simulink model "BESS_PV_WIND_STAGE2_R1_with_scopes_r2024b"  (R2024b)
settings: Solver=VariableStepAuto  StartTime=0.0  StopTime=10.0  RelTol=1e-3
InitFcn:
  | run(fullfile(fileparts(get_param(bdroot,'FileName')),'..','scripts','init_bess_pv_wind_stage2_r1.m'));
undefined symbols (not defined in the file): Control, G, S1, S2, S21, W1
libraries: ee_lib x27, nesl_utility x23, fl_lib x10, simulink x5
(part 1 of 2)
settings Model: Creator=fakebob2004  LastModifiedBy=fakebob2004
settings ModelReferenceCC: UpdateModelReferenceTargets=IfOutOfDate
settings ConfigComp: CovBoundaryAbsTol=1.0e-5
settings SimscapeCC: SimscapeNominalValues="[{\"value\":\"1\",\"unit\":\"A\"},{\"value\":\"1\",\"unit\":\"bar\"},{\"value\":\"1\",\"unit\":\"cm^2\"},{\"value\":\"1\",\"unit\":\"cm^3/s\"},{\"value\":\"1\",\"unit\":\"kJ/kg\"},{\"value\":\"1\",\"unit\":\"kW\"},{\"value\":\"1\",\"unit\":\"l\"},{\"value\":\"1\",\"unit\":\"N\"},{\"value\":\"1\",\"unit\":\"N*m\"},{\"value\":\"1\",\"unit\":\"V\"},{\"value\":\"0.001\",\"unit\":\"Wb\"}]"  SimscapeLogType=all  SimscapeLogDataHistory=10000

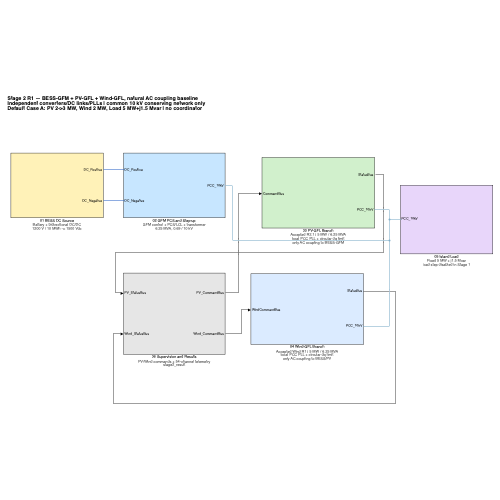
[thumbnail: Simulink's stored preview of the top-level diagram]
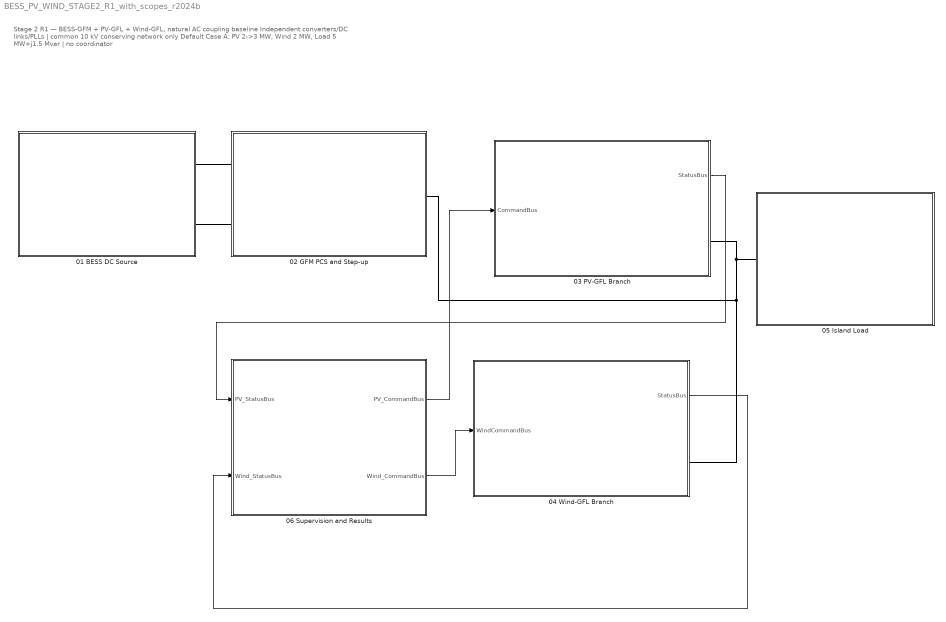
== system BESS_PV_WIND_STAGE2_R1_with_scopes_r2024b ==
  note: Stage 2 R1 — BESS-GFM + PV-GFL + Wind-GFL, natural AC coupling baseline
      | Independent converters/DC links/PLLs | common 10 kV conserving network only
      | Default Case A: PV 2->3 MW, Wind 2 MW, Load 5 MW+j1.5 Mvar | no coordinator
  01 BESS DC Source : Subsystem
      settings: AttributesFormatString=Battery + bidirectional DC/DC\n1200 V / 10 MWh -> 1500 Vdc
  02 GFM PCS and Step-up : Subsystem
      settings: AttributesFormatString=GFM control + PCS/LCL + transformer\n6.25 MVA, 0.69 / 10 kV
  03 PV-GFL Branch : Subsystem
      settings: AttributesFormatString=|
      | Accepted R2.1 | 5 MW / 6.25 MVA
      | local PCC PLL + circular dq limit
      | only AC coupling to BESS-GFM
  04 Wind-GFL Branch : Subsystem
      settings: AttributesFormatString=|
      | Accepted Wind R1 | 5 MW / 6.25 MVA
      | local PCC PLL + circular dq limit
      | only AC coupling to BESS/PV
  05 Island Load : Subsystem
      settings: AttributesFormatString=Fixed 5 MW + j1.5 Mvar\nload step disabled in Stage 1
  06 Supervision and Results : Subsystem
      settings: AttributesFormatString=PV/Wind commands + 54-channel telemetry\nstage2_result
  wires:
  06 Supervision and Results/1(PV_CommandBus) -> 03 PV-GFL Branch/1(CommandBus)
  03 PV-GFL Branch/1(StatusBus) -> 06 Supervision and Results/1(PV_StatusBus)
  06 Supervision and Results/2(Wind_CommandBus) -> 04 Wind-GFL Branch/1(WindCommandBus)
  04 Wind-GFL Branch/1(StatusBus) -> 06 Supervision and Results/2(Wind_StatusBus)
  connections:
  01 BESS DC Source/RConn1 -- 02 GFM PCS and Step-up/LConn1
  01 BESS DC Source/RConn2 -- 02 GFM PCS and Step-up/LConn2
  02 GFM PCS and Step-up/RConn1 -- 04 Wind-GFL Branch/RConn1 -- 05 Island Load/LConn1 -- 03 PV-GFL Branch/RConn1

== system BESS_PV_WIND_STAGE2_R1_with_scopes_r2024b/01 BESS DC Source ==
  01 Battery and DC Link : Subsystem
      settings: AttributesFormatString=1200 V / 10 MWh\n1500 V DC link
  02 Bidirectional DC-DC Control : Subsystem
      settings: AttributesFormatString=Vdc PI: 10 Hz\nIbat PI: 300 Hz
  DC_Positive : PMIOPort  Side=Right  ConnectionType=Connection: foundation.electrical.electrical
  DC_Negative : PMIOPort  Port=2  Side=Right  ConnectionType=Connection: foundation.electrical.electrical
  connections:
  01 Battery and DC Link/RConn1 -- DC_Negative/RConn1
  DC_Positive/RConn1 -- 01 Battery and DC Link/LConn1
  02 Bidirectional DC-DC Control/RConn1 -- 01 Battery and DC Link/LConn2

== system BESS_PV_WIND_STAGE2_R1_with_scopes_r2024b/02 GFM PCS and Step-up ==
  03 GFM Control and Limits : Subsystem
      settings: AttributesFormatString=P-f / Q-V / Virtual Z\nAC limit: 1.20 pu
  04 PCS Filter and Transformer : Subsystem
      settings: AttributesFormatString=6.25 MVA PCS + LCL\n0.69 / 10 kV transformer
  DC_Positive : PMIOPort  Side=Left  ConnectionType=Connection: foundation.electrical.electrical
  DC_Negative : PMIOPort  Port=2  Side=Left  ConnectionType=Connection: foundation.electrical.electrical
  PCC_10kV : PMIOPort  Port=3  Side=Right  ConnectionType=Connection: foundation.electrical.three_phase
  connections:
  04 PCS Filter and Transformer/RConn3 -- DC_Negative/RConn1
  04 PCS Filter and Transformer/RConn2 -- PCC_10kV/RConn1
  04 PCS Filter and Transformer/RConn1 -- DC_Positive/RConn1
  03 GFM Control and Limits/RConn1 -- 04 PCS Filter and Transformer/LConn1

== system BESS_PV_WIND_STAGE2_R1_with_scopes_r2024b/03 PV-GFL Branch ==
  CommandBus : Inport
  01 GFL PCS : Subsystem
  02 Step-up and PCC : Subsystem
  scope_R21_CurrentCommandBus : GotoTagVisibility  GotoTag=R21_CurrentCommandBus
  scope_R21_PCCMeasurementBus : GotoTagVisibility  GotoTag=R21_PCCMeasurementBus
  scope_R21_PrimaryMeasurementBus : GotoTagVisibility  GotoTag=R21_PrimaryMeasurementBus
  PCC_10kV : PMIOPort  Side=Right  ConnectionType=Connection: foundation.electrical.three_phase
  StatusBus : Outport
  wires:
  01 GFL PCS/1(StatusBus) -> StatusBus/1
  CommandBus/1 -> 01 GFL PCS/1(CommandBus)
  connections:
  01 GFL PCS/RConn1 -- 02 Step-up and PCC/LConn1
  02 Step-up and PCC/RConn1 -- PCC_10kV/RConn1

== system BESS_PV_WIND_STAGE2_R1_with_scopes_r2024b/04 Wind-GFL Branch ==
  WindCommandBus : Inport
  01 Aerodynamic and MPPT Available Power : Subsystem
  02 DC Energy Buffer and MSC Equivalent : Subsystem
  03 GFL PCS : Subsystem
  04 Step-up and PCC : Subsystem
  Wind StatusBus Elements : Mux  Inputs=2
  scope_WIND1_CurrentCommandBus : GotoTagVisibility  GotoTag=WIND1_CurrentCommandBus
  scope_WIND1_PCCMeasurementBus : GotoTagVisibility  GotoTag=WIND1_PCCMeasurementBus
  scope_WIND1_PrimaryMeasurementBus : GotoTagVisibility  GotoTag=WIND1_PrimaryMeasurementBus
  PCC_10kV : PMIOPort  Side=Right  ConnectionType=Connection: foundation.electrical.three_phase
  StatusBus : Outport
  wires:
  WindCommandBus/1 -> 01 Aerodynamic and MPPT Available Power/1(WindCommandBus)
  01 Aerodynamic and MPPT Available Power/1(WindSourceBus Out) -> 02 DC Energy Buffer and MSC Equivalent/1(WindSourceBus)
  Wind StatusBus Elements/1 -> StatusBus/1
  02 DC Energy Buffer and MSC Equivalent/1(PCS CommandBus Out) -> 03 GFL PCS/1(CommandBus)
  02 DC Energy Buffer and MSC Equivalent/2(Source StatusBus Out) -> Wind StatusBus Elements/2
  03 GFL PCS/1(StatusBus) -> Wind StatusBus Elements/1
  connections:
  04 Step-up and PCC/RConn1 -- PCC_10kV/RConn1
  03 GFL PCS/RConn1 -- 04 Step-up and PCC/LConn1

== system BESS_PV_WIND_STAGE2_R1_with_scopes_r2024b/05 Island Load ==
  Adjusted_Island_Load : ee_lib/Passive/Constant Power Load (Three-Phase)  port_option=ee.enum.threePhasePort.composite  FRated=G.f0_Hz Hz  active_power=S2.load.base_P_W W  reactive_power=S2.load.base_Q_var V*A  Vline_rms_min=0.70*G.ac.Vll_high_V V  tau=0.01 s  Vline_rms_ini=G.ac.Vll_high_V V  Vang_ini=0 deg  gmin=1e-6 S
  Load_Step_Command : Step  Time=G.load.step_time_s  Before=1  After=0  SampleTime=0
  Load_Step_to_PS : nesl_utility/Simulink-PS Converter  PhysicalDomain=network_engine_domain  SubClassName=ps_input  LeftPortType=input  RightPortType=output  PseudoPeriodic=off  Frequencies=[]  NoiseDistribution=none  NoiseParameters=[]  Unit=V  AffineConversion=off  FilteringAndDerivatives=zero  SimscapeFilterOrder=1  InputFilterTimeConstant=0.001  UdotUserProvided=0
  One_MW_Step_Load : ee_lib/Passive/Constant Power Load (Three-Phase)  port_option=ee.enum.threePhasePort.composite  FRated=G.f0_Hz Hz  active_power=0 W  reactive_power=0 V*A  Vline_rms_min=0.70*G.ac.Vll_high_V V  tau=0.01 s  Vline_rms_ini=G.ac.Vll_high_V V  Vang_ini=0 deg  gmin=1e-6 S
  Step_Load_Breaker : ee_lib/Switches & Breakers/Circuit Breaker (Three-Phase)  port_option=ee.enum.threePhasePort.composite  control_port_option=ee.enum.controlport.ps  R_closed=0.001 Ohm  G_open=1e-6 1/Ohm  threshold=0.5 V  breaker_behavior=ee.enum.switches.breakerBehavior.zeroCrossingEnable  i_th=1e-8 A
  PCC_10kV : PMIOPort  Side=Left  ConnectionType=Connection: foundation.electrical.three_phase
  tag scope: R8_05_Island_Load_Scenario_p1_signal=global
  wires:
  Load_Step_Command/1 -> Load_Step_to_PS/1, [R8_05_Island_Load_Scenario_p1_signal]  "step_breaker_cmd"
  connections:
  Step_Load_Breaker/RConn1 -- One_MW_Step_Load/LConn1
  PCC_10kV/RConn1 -- Adjusted_Island_Load/LConn1 -- Step_Load_Breaker/LConn2
  Load_Step_to_PS/RConn1 -- Step_Load_Breaker/LConn1

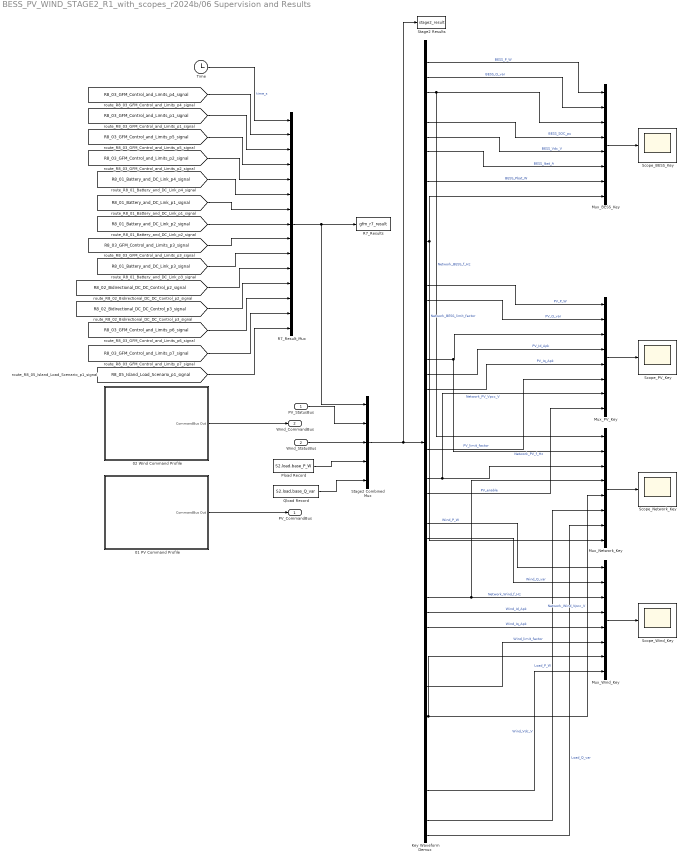
== system BESS_PV_WIND_STAGE2_R1_with_scopes_r2024b/06 Supervision and Results ==
  PV_StatusBus : Inport
  Wind_StatusBus : Inport  Port=2
  01 PV Command Profile : Subsystem
      settings: AttributesFormatString=|
      | CommandBus = [P*, Q*, enable]
      | commissioning scenario only
  02 Wind Command Profile : Subsystem
      settings: AttributesFormatString=|
      | WindCommandBus = [Pavailable, Pdispatch, Q, enable]
      | standalone commissioning scenario only
  Key Waveform Demux : Demux  Outputs=54
  Mux_BESS_Key : Mux  Inputs=8
  Mux_Network_Key : Mux  Inputs=8
  Mux_PV_Key : Mux  Inputs=8
  Mux_Wind_Key : Mux  Inputs=8
  Pload Record : Constant  Value=S2.load.base_P_W
  Qload Record : Constant  Value=S2.load.base_Q_var
  R7_Result_Mux : Mux  Inputs=15
  R7_Results : ToWorkspace  VariableName=gfm_r7_result  SampleTime=-1
  Scope_BESS_Key : Scope
  Scope_Network_Key : Scope
  Scope_PV_Key : Scope
  Scope_Wind_Key : Scope
  Stage2 Combined Mux : Mux  Inputs=5
  Stage2 Results : ToWorkspace  VariableName=stage2_result  SampleTime=-1
  Time : Clock
  PV_CommandBus : Outport
  Wind_CommandBus : Outport  Port=2
  wires:
  [R8_02_Bidirectional_DC_DC_Control_p3_signal] -> R7_Result_Mux/12
  [R8_03_GFM_Control_and_Limits_p4_signal] -> R7_Result_Mux/2
  [R8_01_Battery_and_DC_Link_p2_signal] -> R7_Result_Mux/8
  [R8_02_Bidirectional_DC_DC_Control_p2_signal] -> R7_Result_Mux/11
  [R8_03_GFM_Control_and_Limits_p3_signal] -> R7_Result_Mux/9
  [R8_01_Battery_and_DC_Link_p1_signal] -> R7_Result_Mux/7
  Time/1 -> R7_Result_Mux/1  "time_s"
  [R8_03_GFM_Control_and_Limits_p2_signal] -> R7_Result_Mux/5
  [R8_01_Battery_and_DC_Link_p4_signal] -> R7_Result_Mux/6
  [R8_01_Battery_and_DC_Link_p3_signal] -> R7_Result_Mux/10
  [R8_03_GFM_Control_and_Limits_p1_signal] -> R7_Result_Mux/3
  [R8_03_GFM_Control_and_Limits_p5_signal] -> R7_Result_Mux/4
  [R8_03_GFM_Control_and_Limits_p6_signal] -> R7_Result_Mux/13
  [R8_03_GFM_Control_and_Limits_p7_signal] -> R7_Result_Mux/14
  02 Wind Command Profile/1(CommandBus Out) -> Wind_CommandBus/1
  [R8_05_Island_Load_Scenario_p1_signal] -> R7_Result_Mux/15
  Key Waveform Demux/54 -> Mux_Network_Key/7  "Load_Q_var"
  Key Waveform Demux/46 -> Mux_Wind_Key/7, Mux_Network_Key/5  "Network_Wind_Vpcc_V"
  Key Waveform Demux/38 -> Mux_Wind_Key/3, Mux_Network_Key/4  "Network_Wind_f_Hz"
  01 PV Command Profile/1(CommandBus Out) -> PV_CommandBus/1
  Pload Record/1 -> Stage2 Combined Mux/4
  R7_Result_Mux/1 -> Stage2 Combined Mux/1, R7_Results/1
  Key Waveform Demux/39 -> Mux_Wind_Key/4  "Wind_Id_Apk"
  Key Waveform Demux/31 -> Mux_PV_Key/8  "PV_enable"
  PV_StatusBus/1 -> Stage2 Combined Mux/2
  Wind_StatusBus/1 -> Stage2 Combined Mux/3
  Qload Record/1 -> Stage2 Combined Mux/5
  Stage2 Combined Mux/1 -> Key Waveform Demux/1, Stage2 Results/1
  Key Waveform Demux/18 -> Mux_PV_Key/2  "PV_Q_var"
  Key Waveform Demux/10 -> Mux_BESS_Key/7  "BESS_Pbat_W"
  Key Waveform Demux/2 -> Mux_BESS_Key/1  "BESS_P_W"
  Key Waveform Demux/3 -> Mux_BESS_Key/2  "BESS_Q_var"
  Key Waveform Demux/28 -> Mux_PV_Key/6  "PV_limit_factor"
  Key Waveform Demux/4 -> Mux_BESS_Key/3, Mux_Network_Key/1  "Network_BESS_f_Hz"
  Key Waveform Demux/30 -> Mux_PV_Key/7, Mux_Network_Key/3  "Network_PV_Vpcc_V"
  Key Waveform Demux/22 -> Mux_PV_Key/3, Mux_Network_Key/2  "Network_PV_f_Hz"
  Key Waveform Demux/14 -> Mux_BESS_Key/8, Mux_Network_Key/8  "Network_BESS_limit_factor"
  Key Waveform Demux/6 -> Mux_BESS_Key/4  "BESS_SOC_pu"
  Key Waveform Demux/23 -> Mux_PV_Key/4  "PV_Id_Apk"
  Key Waveform Demux/7 -> Mux_BESS_Key/5  "BESS_Vdc_V"
  Key Waveform Demux/24 -> Mux_PV_Key/5  "PV_Iq_Apk"
  Key Waveform Demux/8 -> Mux_BESS_Key/6  "BESS_Ibat_A"
  Key Waveform Demux/17 -> Mux_PV_Key/1  "PV_P_W"
  Key Waveform Demux/33 -> Mux_Wind_Key/1  "Wind_P_W"
  Key Waveform Demux/34 -> Mux_Wind_Key/2  "Wind_Q_var"
  Key Waveform Demux/40 -> Mux_Wind_Key/5  "Wind_Iq_Apk"
  Mux_BESS_Key/1 -> Scope_BESS_Key/1
  Key Waveform Demux/44 -> Mux_Wind_Key/6  "Wind_limit_factor"
  Key Waveform Demux/51 -> Mux_Wind_Key/8  "Wind_Vdc_V"
  Key Waveform Demux/53 -> Mux_Network_Key/6  "Load_P_W"
  Mux_PV_Key/1 -> Scope_PV_Key/1
  Mux_Network_Key/1 -> Scope_Network_Key/1
  Mux_Wind_Key/1 -> Scope_Wind_Key/1

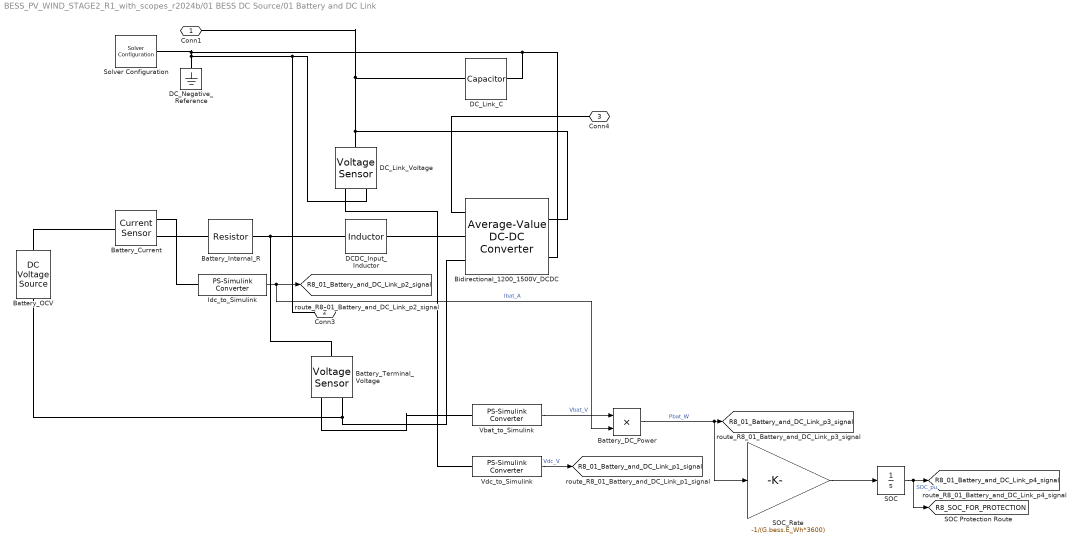
== system BESS_PV_WIND_STAGE2_R1_with_scopes_r2024b/01 BESS DC Source/01 Battery and DC Link ==
  Battery_Current : fl_lib/Electrical/Electrical Sensors/Current Sensor
  Battery_DC_Power : Product
  Battery_Internal_R : fl_lib/Electrical/Electrical Elements/Resistor  R=G.dc.Rbattery_ohm Ohm  i_specify=off  i_priority=None  i=0 A  i_nominal_specify=off  i_nominal_value=1  i_nominal_unit=A  v_specify=off  v_priority=None  v=0 V  v_nominal_specify=off  v_nominal_value=1  v_nominal_unit=V
  Battery_OCV : fl_lib/Electrical/Electrical Sources/DC Voltage Source  v0=G.dc.Vbattery_V V
  Battery_Terminal_Voltage : fl_lib/Electrical/Electrical Sensors/Voltage Sensor
  Bidirectional_1200_1500V_DCDC : ee_lib/Semiconductors & Converters/Converters/Average-Value DC-DC Converter  implementation_option=ee.enum.converters.implementation.behavioral  converter_type=ee.enum.converters.dcdctype.buckboost  control_option=ee.enum.converters.controlinput.dutycycle  efficiency_option=ee.enum.converters.efficiency.constant  efficiency_fixed=G.dc.dcdc_efficiency_pct  i_vec=[0, 2, 5] A  efficiency_vec=[90, 95, 98]  Lf=1e-6 H  Rl=0 Ohm  Cf=1e-7 F  Rc=1e-6 Ohm  iL_specify=off  iL_priority=High  iL=0 A  iL_nominal_specify=off  iL_nominal_value=1  iL_nominal_unit=A  vc_specify=off  vc_priority=High  vc=0 V  vc_nominal_specify=off  vc_nominal_value=1  vc_nominal_unit=V
  DCDC_Input_Inductor : fl_lib/Electrical/Electrical Elements/Inductor  l=G.dcdc.L_H H  r=0 Ohm  g=1e-9 1/Ohm  i_specify=on  i_priority=None  i=G.dcdc.Iref_initial_A A  i_nominal_specify=off  i_nominal_value=1  i_nominal_unit=A  v_specify=off  v_priority=None  v=0 V  v_nominal_specify=off  v_nominal_value=1  v_nominal_unit=V  i_L_specify=off  i_L_priority=High  i_L=0 A  i_L_nominal_specify=off  i_L_nominal_value=1  i_L_nominal_unit=A
  DC_Link_C : fl_lib/Electrical/Electrical Elements/Capacitor  c=G.dc.Cdc_F F  r=1e-6 Ohm  g=0 1/Ohm  i_specify=off  i_priority=None  i=0 A  i_nominal_specify=off  i_nominal_value=1  i_nominal_unit=A  v_specify=off  v_priority=None  v=0 V  v_nominal_specify=off  v_nominal_value=1  v_nominal_unit=V  vc_specify=on  vc_priority=High  vc=G.dc.Vdc_ref_V V  vc_nominal_specify=off  vc_nominal_value=1  vc_nominal_unit=V
  DC_Link_Voltage : fl_lib/Electrical/Electrical Sensors/Voltage Sensor
  DC_Negative_Reference : fl_lib/Electrical/Electrical Elements/Electrical Reference
  Idc_to_Simulink : nesl_utility/PS-Simulink Converter  PhysicalDomain=network_engine_domain  SubClassName=ps_output  LeftPortType=input  RightPortType=output  PseudoPeriodic=off  Frequencies=[]  VectorFormat=inherit  Unit=A  AffineConversion=off
  SOC : Integrator  InitialCondition=G.bess.SOC0  LimitOutput=on  UpperSaturationLimit=G.bess.SOC_max  LowerSaturationLimit=G.bess.SOC_min
  SOC_Rate : Gain  Gain=-1/(G.bess.E_Wh*3600)
  Solver Configuration : nesl_utility/Solver Configuration  PhysicalDomain=network_engine_domain  SubClassName=solver  LeftPortType=input  RightPortType=generic  Tones=[]  Harmonics=[]  SimulateNoise=off  Profile=off  UseLocalSampling=off  EnableSwitchedLinearOptims=on  FrequencyDomain=off  UseCCode=off  RelTol=0.001  AbsTol=0.001  MinStep=1e-09  ToWorkspace=off  RevertToSquareIcSolve=off  NumHomotopyIterations=100  PhasorMode=off  PhasorModeNumHarmonics=1  ConsistencySolver=NEWTON_XTOL_AFTER_FTOL  CanonicalOrdering=CANONICAL  OptimizeIntermediates=OPTIMIZED  IndexReductionMethod=DerivativeReplacement  DoDC=off  ResidualTolerance=1e-09  ConsistencyTolSource=GLOBAL  ConsistencyAbsTol=0.001  ConsistencyRelTol=0.001  ConsistencyTolFactor=0.001  UseLocalSolver=off  LocalSolverChoice=NE_BACKWARD_EULER_ADVANCER  ResolveIndetEquations=on  FunctionEvalNumThread=1  LocalSolverSampleTime=0.001  DoFixedCost=off  MaxNonlinIter=3  MaxModeIter=2  ComputeImpulses=off  ImpulseIterations=2  LinearAlgebra=auto  LinearAlgebraNumThread=0  EquationFormulation=NE_TIME_EF  DelaysMemoryBudget=1024  AutomaticFiltering=on  FilteringTimeConstant=0.001  PartitionStorageMethod=AS_NEEDED  PartitionMemoryBudget=1024  PartitionMethod=ROBUST  MultibodyUseLocalSolver=off  MultibodyLocalSolverChoice=ODE1  MultibodyLocalSolverSampleTime=0.001
  Vbat_to_Simulink : nesl_utility/PS-Simulink Converter  PhysicalDomain=network_engine_domain  SubClassName=ps_output  LeftPortType=input  RightPortType=output  PseudoPeriodic=off  Frequencies=[]  VectorFormat=inherit  Unit=V  AffineConversion=off
  Vdc_to_Simulink : nesl_utility/PS-Simulink Converter  PhysicalDomain=network_engine_domain  SubClassName=ps_output  LeftPortType=input  RightPortType=output  PseudoPeriodic=off  Frequencies=[]  VectorFormat=inherit  Unit=V  AffineConversion=off
  Conn1 : PMIOPort  Side=Left
  Conn3 : PMIOPort  Port=2  Side=Right
  Conn4 : PMIOPort  Port=3  Side=Left
  tag scope: R8_01_Battery_and_DC_Link_p1_signal=global, R8_01_Battery_and_DC_Link_p2_signal=global, R8_01_Battery_and_DC_Link_p3_signal=global, R8_01_Battery_and_DC_Link_p4_signal=global, R8_SOC_FOR_PROTECTION=global
  wires:
  Idc_to_Simulink/1 -> [R8_01_Battery_and_DC_Link_p2_signal], Battery_DC_Power/2  "Ibat_A"
  SOC_Rate/1 -> SOC/1
  Vbat_to_Simulink/1 -> Battery_DC_Power/1  "Vbat_V"
  SOC/1 -> [R8_SOC_FOR_PROTECTION], [R8_01_Battery_and_DC_Link_p4_signal]  "SOC_pu"
  Vdc_to_Simulink/1 -> [R8_01_Battery_and_DC_Link_p1_signal]  "Vdc_V"
  Battery_DC_Power/1 -> [R8_01_Battery_and_DC_Link_p3_signal], SOC_Rate/1  "Pbat_W"
  connections:
  Battery_Internal_R/RConn1 -- Battery_Terminal_Voltage/LConn1 -- DCDC_Input_Inductor/LConn1
  Battery_Current/RConn1 -- Idc_to_Simulink/LConn1
  Battery_Terminal_Voltage/RConn1 -- Vbat_to_Simulink/LConn1
  Battery_OCV/LConn1 -- Battery_Current/LConn1
  Battery_OCV/RConn1 -- Battery_Terminal_Voltage/RConn2 -- Bidirectional_1200_1500V_DCDC/LConn3
  Battery_Current/RConn2 -- Battery_Internal_R/LConn1
  DC_Negative_Reference/LConn1 -- DC_Link_Voltage/RConn2 -- Conn3/RConn1 -- DC_Link_C/RConn1 -- Bidirectional_1200_1500V_DCDC/RConn2 -- Solver Configuration/RConn1
  DC_Link_Voltage/RConn1 -- Vdc_to_Simulink/LConn1
  DC_Link_Voltage/LConn1 -- Conn1/RConn1 -- DC_Link_C/LConn1 -- Bidirectional_1200_1500V_DCDC/RConn1
  DCDC_Input_Inductor/RConn1 -- Bidirectional_1200_1500V_DCDC/LConn2
  Conn4/RConn1 -- Bidirectional_1200_1500V_DCDC/LConn1

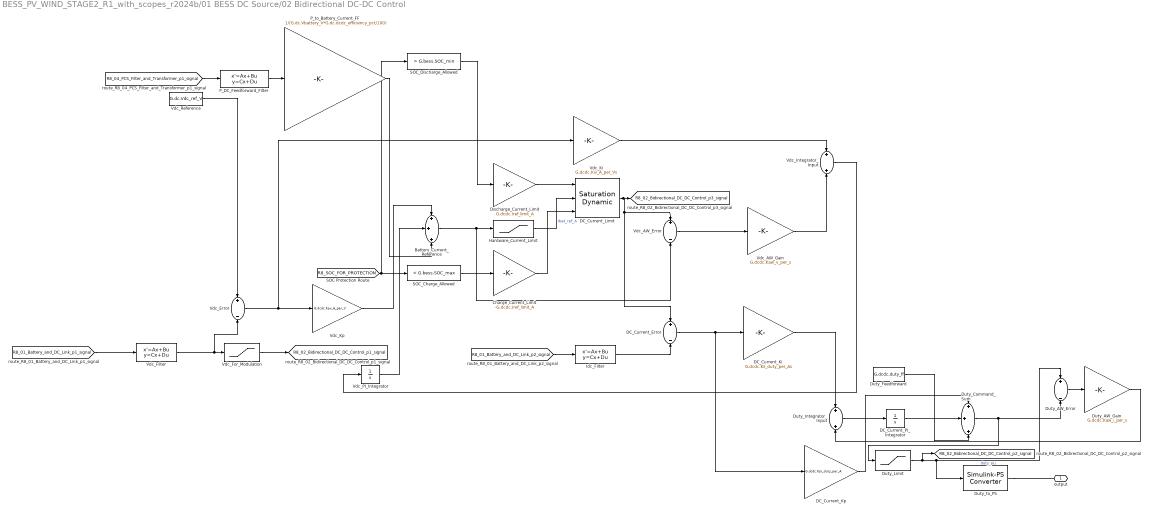
== system BESS_PV_WIND_STAGE2_R1_with_scopes_r2024b/01 BESS DC Source/02 Bidirectional DC-DC Control ==
  Battery_Current_Reference : Sum  Inputs=+++
  Charge_Current_Limit : Gain  Gain=-G.dcdc.Iref_limit_A
  DC_Current_Error : Sum  Inputs=+-
  DC_Current_Ki : Gain  Gain=G.dcdc.Kii_duty_per_As
  DC_Current_Kp : Gain  Gain=G.dcdc.Kpi_duty_per_A
  DC_Current_Limit : simulink/Discontinuities/Saturation Dynamic  OutMin=[]  OutMax=[]  OutDataTypeStr=Inherit: Same as second input  OutDataType=fixdt(1, 16)  OutScaling=2^-10  DoSatur=off
      settings: LibrarySourceBlock=|
      | simulink/Discontinuities/Saturation
      | Dynamic
  DC_Current_PI_Integrator : Integrator
  Discharge_Current_Limit : Gain  Gain=G.dcdc.Iref_limit_A
  Duty_AW_Error : Sum  Inputs=+-
  Duty_AW_Gain : Gain  Gain=G.dcdc.Kaw_i_per_s
  Duty_Command_Sum : Sum  Inputs=+++
  Duty_Feedforward : Constant  Value=G.dcdc.duty_ff
  Duty_Integrator_Input : Sum
  Duty_Limit : Saturate  UpperLimit=G.dcdc.duty_max  LowerLimit=G.dcdc.duty_min
  Duty_to_PS : nesl_utility/Simulink-PS Converter  PhysicalDomain=network_engine_domain  SubClassName=ps_input  LeftPortType=input  RightPortType=output  PseudoPeriodic=off  Frequencies=[]  NoiseDistribution=none  NoiseParameters=[]  Unit=1  AffineConversion=off  FilteringAndDerivatives=zero  SimscapeFilterOrder=1  InputFilterTimeConstant=0.001  UdotUserProvided=0
  Hardware_Current_Limit : Saturate  UpperLimit=G.dcdc.Iref_limit_A  LowerLimit=-G.dcdc.Iref_limit_A
  Idc_Filter : StateSpace  A=-1/G.dcdc.current_sensor_s  B=1/G.dcdc.current_sensor_s  D=0  InitialCondition=G.dcdc.Iref_initial_A
  P_DC_Feedforward_Filter : StateSpace  A=-1/G.dcdc.power_ff_filter_s  B=1/G.dcdc.power_ff_filter_s  D=0  InitialCondition=G.load.base_P_W
  P_to_Battery_Current_FF : Gain  Gain=1/(G.dc.Vbattery_V*G.dc.dcdc_efficiency_pct/100)
  SOC_Charge_Allowed : simulink/Logic and Bit Operations/Compare To Constant  relop=<  const=G.bess.SOC_max  OutDataTypeStr=boolean
  SOC_Discharge_Allowed : simulink/Logic and Bit Operations/Compare To Constant  relop=>  const=G.bess.SOC_min  OutDataTypeStr=boolean
  Vdc_AW_Error : Sum  Inputs=+-
  Vdc_AW_Gain : Gain  Gain=G.dcdc.Kaw_v_per_s
  Vdc_Error : Sum  Inputs=+-
  Vdc_Filter : StateSpace  A=-1/G.control.Vdc_filter_s  B=1/G.control.Vdc_filter_s  D=0  InitialCondition=G.dc.Vdc_ref_V
  Vdc_For_Modulation : Saturate  UpperLimit=2000  LowerLimit=500
  Vdc_Integrator_Input : Sum
  Vdc_Ki : Gain  Gain=G.dcdc.Kiv_A_per_Vs
  Vdc_Kp : Gain  Gain=G.dcdc.Kpv_A_per_V
  Vdc_PI_Integrator : Integrator
  Vdc_Reference : Constant  Value=G.dc.Vdc_ref_V
  output : PMIOPort  Side=Right
  tag scope: R8_02_Bidirectional_DC_DC_Control_p1_signal=global, R8_02_Bidirectional_DC_DC_Control_p2_signal=global, R8_02_Bidirectional_DC_DC_Control_p3_signal=global
  wires:
  Vdc_Ki/1 -> Vdc_Integrator_Input/1
  Vdc_Reference/1 -> Vdc_Error/1
  [R8_01_Battery_and_DC_Link_p2_signal] -> Idc_Filter/1
  [R8_04_PCS_Filter_and_Transformer_p1_signal] -> P_DC_Feedforward_Filter/1
  [R8_01_Battery_and_DC_Link_p1_signal] -> Vdc_Filter/1
  Vdc_For_Modulation/1 -> [R8_02_Bidirectional_DC_DC_Control_p1_signal]
  Vdc_AW_Gain/1 -> Vdc_Integrator_Input/2
  Vdc_Error/1 -> Vdc_Ki/1, Vdc_Kp/1
  Vdc_Filter/1 -> Vdc_Error/2, Vdc_For_Modulation/1
  SOC_Discharge_Allowed/1 -> Discharge_Current_Limit/1
  P_to_Battery_Current_FF/1 -> Battery_Current_Reference/3
  SOC_Charge_Allowed/1 -> Charge_Current_Limit/1
  P_DC_Feedforward_Filter/1 -> P_to_Battery_Current_FF/1
  Idc_Filter/1 -> DC_Current_Error/2
  [R8_SOC_FOR_PROTECTION] -> SOC_Charge_Allowed/1, SOC_Discharge_Allowed/1
  Vdc_Kp/1 -> Battery_Current_Reference/1
  Vdc_PI_Integrator/1 -> Battery_Current_Reference/2
  Charge_Current_Limit/1 -> DC_Current_Limit/3
  Battery_Current_Reference/1 -> Vdc_AW_Error/2, Hardware_Current_Limit/1
  Duty_AW_Error/1 -> Duty_AW_Gain/1
  Discharge_Current_Limit/1 -> DC_Current_Limit/1
  Hardware_Current_Limit/1 -> DC_Current_Limit/2  "Ibat_ref_A"
  DC_Current_Ki/1 -> Duty_Integrator_Input/1
  DC_Current_Limit/1 -> Vdc_AW_Error/1, DC_Current_Error/1, [R8_02_Bidirectional_DC_DC_Control_p3_signal]
  Vdc_AW_Error/1 -> Vdc_AW_Gain/1
  DC_Current_Error/1 -> DC_Current_Kp/1, DC_Current_Ki/1
  Vdc_Integrator_Input/1 -> Vdc_PI_Integrator/1
  Duty_Feedforward/1 -> Duty_Command_Sum/3
  Duty_Integrator_Input/1 -> DC_Current_PI_Integrator/1
  DC_Current_PI_Integrator/1 -> Duty_Command_Sum/2
  DC_Current_Kp/1 -> Duty_Command_Sum/1
  Duty_Limit/1 -> Duty_AW_Error/1, Duty_to_PS/1, [R8_02_Bidirectional_DC_DC_Control_p2_signal]  "duty_pu"
  Duty_AW_Gain/1 -> Duty_Integrator_Input/2
  Duty_Command_Sum/1 -> Duty_AW_Error/2, Duty_Limit/1
  connections:
  Duty_to_PS/RConn1 -- output/RConn1

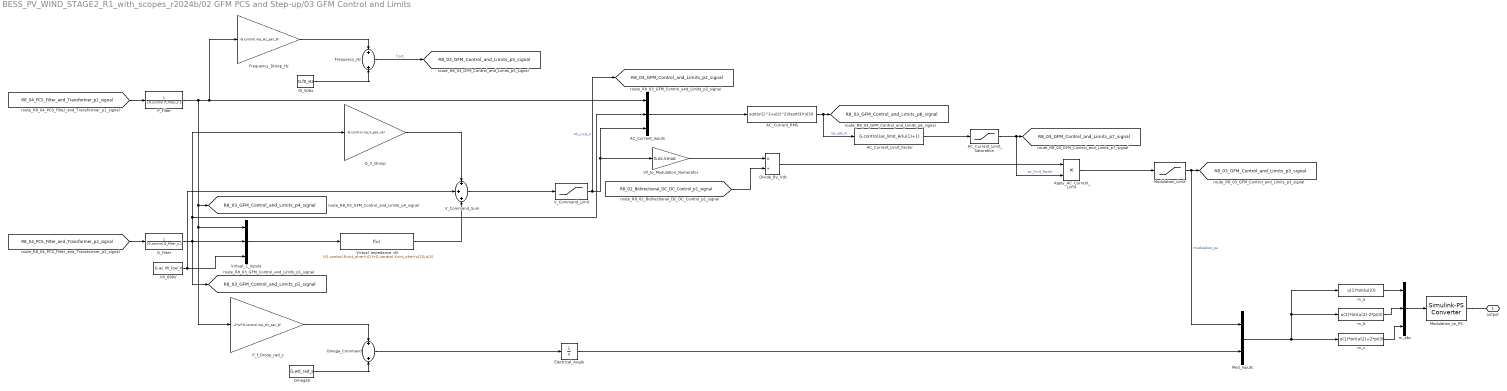
== system BESS_PV_WIND_STAGE2_R1_with_scopes_r2024b/02 GFM PCS and Step-up/03 GFM Control and Limits ==
  AC_Current_Inputs : Mux  Inputs=3
  AC_Current_Limit_Factor : Fcn  Expr=G.control.Iac_limit_A/(u(1)+1)
  AC_Current_Limit_Saturation : Saturate  UpperLimit=1  LowerLimit=0
  AC_Current_RMS : Fcn  Expr=sqrt(u(1)^2+u(2)^2)/(sqrt(3)*u(3))
  Apply_AC_Current_Limit : Product
  Divide_By_Vdc : Product  Inputs=*/
  Electrical_Angle : Integrator  InitialCondition=pi/6
  Frequency_Droop_Hz : Gain  Gain=-G.control.mp_Hz_per_W
  Frequency_Hz : Sum
  Mod_Inputs : Mux  Inputs=2
  Modulation_Limit : Saturate  UpperLimit=G.dc.modulation_max  LowerLimit=0
  Modulation_to_PS : nesl_utility/Simulink-PS Converter  PhysicalDomain=network_engine_domain  SubClassName=ps_input  LeftPortType=input  RightPortType=output  PseudoPeriodic=off  Frequencies=[]  NoiseDistribution=none  NoiseParameters=[]  Unit=1  AffineConversion=off  FilteringAndDerivatives=zero  SimscapeFilterOrder=1  InputFilterTimeConstant=0.001  UdotUserProvided=0
  Omega0 : Constant  Value=G.w0_rad_s
  Omega_Command : Sum
  P_Filter : TransferFcn  Numerator=1  Denominator=[G.control.P_filter_s 1]
  P_f_Droop_rad_s : Gain  Gain=-2*pi*G.control.mp_Hz_per_W
  Q_Filter : TransferFcn  Numerator=1  Denominator=[G.control.Q_filter_s 1]
  Q_V_Droop : Gain  Gain=-G.control.nq_V_per_var
  V0_690V : Constant  Value=G.ac.Vll_low_V
  V_Command_Limit : Saturate  UpperLimit=1.10*G.ac.Vll_low_V  LowerLimit=0.90*G.ac.Vll_low_V
  V_Command_Sum : Sum  Inputs=+++
  Virtual_Impedance_dV : Fcn  Expr=(-G.control.Rvirt_ohm*u(1)+G.control.Xvirt_ohm*u(2))/u(3)
  Virtual_Z_Inputs : Mux  Inputs=3
  Vll_to_Modulation_Numerator : Gain  Gain=G.dc.kmod
  f0_50Hz : Constant  Value=G.f0_Hz
  m_a : Fcn  Expr=u(1)*sin(u(2))
  m_abc : Mux  Inputs=3
  m_b : Fcn  Expr=u(1)*sin(u(2)-2*pi/3)
  m_c : Fcn  Expr=u(1)*sin(u(2)+2*pi/3)
  output : PMIOPort  Side=Right
  tag scope: R8_03_GFM_Control_and_Limits_p1_signal=global, R8_03_GFM_Control_and_Limits_p2_signal=global, R8_03_GFM_Control_and_Limits_p3_signal=global, R8_03_GFM_Control_and_Limits_p4_signal=global, R8_03_GFM_Control_and_Limits_p5_signal=global, R8_03_GFM_Control_and_Limits_p6_signal=global, R8_03_GFM_Control_and_Limits_p7_signal=global
  wires:
  [R8_04_PCS_Filter_and_Transformer_p2_signal] -> Q_Filter/1
  [R8_02_Bidirectional_DC_DC_Control_p1_signal] -> Divide_By_Vdc/2
  [R8_04_PCS_Filter_and_Transformer_p1_signal] -> P_Filter/1
  Mod_Inputs/1 -> m_b/1, m_a/1, m_c/1
  P_f_Droop_rad_s/1 -> Omega_Command/1
  V0_690V/1 -> V_Command_Sum/2, Virtual_Z_Inputs/3
  V_Command_Limit/1 -> Vll_to_Modulation_Numerator/1, AC_Current_Inputs/3, [R8_03_GFM_Control_and_Limits_p2_signal]  "Vll_cmd_V"
  Q_Filter/1 -> Q_V_Droop/1, AC_Current_Inputs/2, Virtual_Z_Inputs/2, [R8_03_GFM_Control_and_Limits_p1_signal]
  P_Filter/1 -> Virtual_Z_Inputs/1, P_f_Droop_rad_s/1, [R8_03_GFM_Control_and_Limits_p4_signal], AC_Current_Inputs/1, Frequency_Droop_Hz/1
  Frequency_Droop_Hz/1 -> Frequency_Hz/1
  Virtual_Z_Inputs/1 -> Virtual_Impedance_dV/1
  f0_50Hz/1 -> Frequency_Hz/2
  Q_V_Droop/1 -> V_Command_Sum/1
  Omega0/1 -> Omega_Command/2
  AC_Current_Limit_Factor/1 -> AC_Current_Limit_Saturation/1
  Frequency_Hz/1 -> [R8_03_GFM_Control_and_Limits_p5_signal]  "f_Hz"
  m_c/1 -> m_abc/3
  Vll_to_Modulation_Numerator/1 -> Divide_By_Vdc/1
  Virtual_Impedance_dV/1 -> V_Command_Sum/3
  Omega_Command/1 -> Electrical_Angle/1
  V_Command_Sum/1 -> V_Command_Limit/1
  Electrical_Angle/1 -> Mod_Inputs/2
  Divide_By_Vdc/1 -> Apply_AC_Current_Limit/1
  AC_Current_RMS/1 -> AC_Current_Limit_Factor/1, [R8_03_GFM_Control_and_Limits_p6_signal]  "Iac_est_A"
  AC_Current_Inputs/1 -> AC_Current_RMS/1
  AC_Current_Limit_Saturation/1 -> Apply_AC_Current_Limit/2, [R8_03_GFM_Control_and_Limits_p7_signal]  "ac_limit_factor"
  Apply_AC_Current_Limit/1 -> Modulation_Limit/1
  Modulation_Limit/1 -> Mod_Inputs/1, [R8_03_GFM_Control_and_Limits_p3_signal]  "modulation_pu"
  m_b/1 -> m_abc/2
  m_a/1 -> m_abc/1
  m_abc/1 -> Modulation_to_PS/1
  connections:
  Modulation_to_PS/RConn1 -- output/RConn1

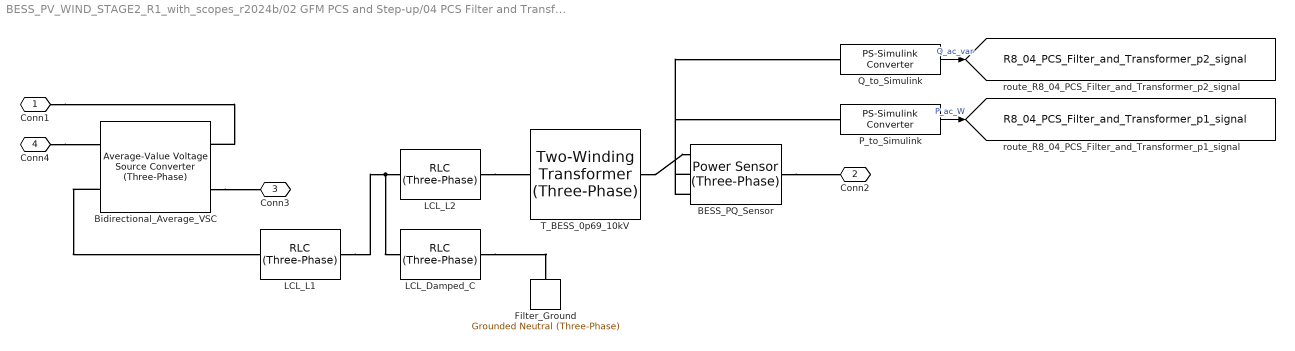
== system BESS_PV_WIND_STAGE2_R1_with_scopes_r2024b/02 GFM PCS and Step-up/04 PCS Filter and Transformer ==
  BESS_PQ_Sensor : ee_lib/Sensors & Transducers/Power Sensor (Three-Phase)  port_option=ee.enum.threePhasePort.composite  load_type=ee.enum.passive.type_balanced.balanced  f0=60 Hz
  Bidirectional_Average_VSC : ee_lib/Semiconductors & Converters/Converters/Average-Value Voltage Source Converter (Three-Phase)  port_option=ee.enum.threePhasePort.composite  enable_block_pulses_input=false  krec=G.dc.Rbattery_ohm/10 Ohm  frequency_option=ee.enum.converters.frequency.variable  input_option=ee.enum.converters.inputOption.ModWave  FRated=G.f0_Hz Hz  losses_parameterization=ee.enum.converters.losses.fixed  Pfixed=1 W  ks=0.01  kc1=1.7 V  kc2=0.01 Ohm  Ploss_vect=[100, 800, 1870, 3250, 4900] W  Irms_vect=[10, 100, 200, 300, 400] A  Vdc_nom=300 V  thermal_mass=30000 J/K  temperature_specify=off  temperature_priority=High  temperature=298.15 K  temperature_nominal_specify=off  temperature_nominal_value=1  temperature_nominal_unit=K
  Filter_Ground : ee_lib/Connectors & References/Grounded Neutral (Three-Phase)  port_option=ee.enum.threePhasePort.composite
  LCL_Damped_C : ee_lib/Passive/RLC Assemblies/RLC (Three-Phase)  port_option=ee.enum.threePhasePort.composite  component_structure=ee.enum.rlc.structure.SeriesRC  R=G.filter.Rd_ohm Ohm  L=1e-3 H  C=G.filter.C_F F  R_parasitic=0 Ohm  G_parasitic=0 1/Ohm  IL_specify=off  IL_priority=High  IL=[0, 0, 0] A  IL_nominal_specify=off  IL_nominal_value=1  IL_nominal_unit=A  VC_specify=off  VC_priority=High  VC=[0, 0, 0] V  VC_nominal_specify=off  VC_nominal_value=1  VC_nominal_unit=V
  LCL_L1 : ee_lib/Passive/RLC Assemblies/RLC (Three-Phase)  port_option=ee.enum.threePhasePort.composite  component_structure=ee.enum.rlc.structure.SeriesRL  R=G.filter.R1_ohm Ohm  L=G.filter.L1_H H  C=1e-6 F  R_parasitic=0 Ohm  G_parasitic=0 1/Ohm  IL_specify=off  IL_priority=High  IL=[0, 0, 0] A  IL_nominal_specify=off  IL_nominal_value=1  IL_nominal_unit=A  VC_specify=off  VC_priority=High  VC=[0, 0, 0] V  VC_nominal_specify=off  VC_nominal_value=1  VC_nominal_unit=V
  LCL_L2 : ee_lib/Passive/RLC Assemblies/RLC (Three-Phase)  port_option=ee.enum.threePhasePort.composite  component_structure=ee.enum.rlc.structure.SeriesRL  R=G.filter.R2_ohm Ohm  L=G.filter.L2_H H  C=1e-6 F  R_parasitic=0 Ohm  G_parasitic=0 1/Ohm  IL_specify=off  IL_priority=High  IL=[0, 0, 0] A  IL_nominal_specify=off  IL_nominal_value=1  IL_nominal_unit=A  VC_specify=off  VC_priority=High  VC=[0, 0, 0] V  VC_nominal_specify=off  VC_nominal_value=1  VC_nominal_unit=V
  P_to_Simulink : nesl_utility/PS-Simulink Converter  PhysicalDomain=network_engine_domain  SubClassName=ps_output  LeftPortType=input  RightPortType=output  PseudoPeriodic=off  Frequencies=[]  VectorFormat=inherit  Unit=W  AffineConversion=off
  Q_to_Simulink : nesl_utility/PS-Simulink Converter  PhysicalDomain=network_engine_domain  SubClassName=ps_output  LeftPortType=input  RightPortType=output  PseudoPeriodic=off  Frequencies=[]  VectorFormat=inherit  Unit=W  AffineConversion=off
  T_BESS_0p69_10kV : ee_lib/Passive/Transformers/Two-Winding Transformer (Three-Phase)  SRated=G.transformer.S_VA A*V  FRated=G.f0_Hz Hz  Winding1Connection=ee.enum.windingconnection.delta1  VRated1=G.ac.Vll_low_V V  Winding2Connection=ee.enum.windingconnection.Yg  VRated2=G.ac.Vll_high_V V  CoreType=ee.enum.coretype.threelimb  pu_Rw1=G.transformer.pu_Rw1  pu_Rw2=G.transformer.pu_Rw2  leakage_reactance_option=ee.enum.transformer_leakage.include  pu_Xl1=G.transformer.pu_Xl1  pu_Xl2=G.transformer.pu_Xl2  magnetizing_resistance_option=ee.enum.transformer_magnetizingResistance.exclude  pu_Rm=500  magnetizing_reactance_option=ee.enum.transformer_magnetizingReactance.exclude  saturation_option=ee.enum.transformer_saturation.exclude  pu_Xm=500  current_data=[0, .002, 1, 2]  magnetic_flux_data=[0, 1.2, 1.5, 1.51]  pu_X0=0.5  i1_specify=off  i1_priority=None  i1=[0, 0, 0] A  i1_nominal_specify=off  i1_nominal_value=1  i1_nominal_unit=A  i2_specify=off  i2_priority=None  i2=[0, 0, 0] A  i2_nominal_specify=off  i2_nominal_value=1  i2_nominal_unit=A  phi_specify=off  phi_priority=None  phi=[0, 0, 0]  phi_nominal_specify=off  phi_nominal_value=1  phi_nominal_unit=1
  Conn1 : PMIOPort  Side=Right  ConnectionType=Connection: foundation.electrical.electrical
  Conn2 : PMIOPort  Port=2  Side=Right  ConnectionType=Connection: foundation.electrical.three_phase
  Conn3 : PMIOPort  Port=3  Side=Right  ConnectionType=Connection: foundation.electrical.electrical
  Conn4 : PMIOPort  Port=4  Side=Left
  tag scope: R8_04_PCS_Filter_and_Transformer_p1_signal=global, R8_04_PCS_Filter_and_Transformer_p2_signal=global
  wires:
  P_to_Simulink/1 -> [R8_04_PCS_Filter_and_Transformer_p1_signal]  "P_ac_W"
  Q_to_Simulink/1 -> [R8_04_PCS_Filter_and_Transformer_p2_signal]  "Q_ac_var"
  connections:
  T_BESS_0p69_10kV/RConn1 -- BESS_PQ_Sensor/LConn1
  LCL_Damped_C/RConn1 -- Filter_Ground/LConn1
  LCL_L2/RConn1 -- T_BESS_0p69_10kV/LConn1
  Conn4/RConn1 -- Bidirectional_Average_VSC/LConn1
  LCL_L1/RConn1 -- LCL_L2/LConn1 -- LCL_Damped_C/LConn1
  Conn1/RConn1 -- Bidirectional_Average_VSC/RConn1
  Bidirectional_Average_VSC/RConn2 -- Conn3/RConn1
  Bidirectional_Average_VSC/LConn2 -- LCL_L1/LConn1
  BESS_PQ_Sensor/RConn1 -- Conn2/RConn1
  BESS_PQ_Sensor/LConn2 -- P_to_Simulink/LConn1
  BESS_PQ_Sensor/LConn3 -- Q_to_Simulink/LConn1

== system BESS_PV_WIND_STAGE2_R1_with_scopes_r2024b/03 PV-GFL Branch/01 GFL PCS ==
  CommandBus : Inport
  01 Secondary Control : Subsystem
  02 Primary Converter and Filter : Subsystem
  AC_690V : PMIOPort  Side=Right
  StatusBus : Outport
  wires:
  01 Secondary Control/4(Out4) -> StatusBus/1
  CommandBus/1 -> 01 Secondary Control/1(In1)
  connections:
  02 Primary Converter and Filter/RConn1 -- AC_690V/RConn1

== system BESS_PV_WIND_STAGE2_R1_with_scopes_r2024b/03 PV-GFL Branch/02 Step-up and PCC ==
  P to Simulink : nesl_utility/PS-Simulink Converter  PhysicalDomain=network_engine_domain  SubClassName=ps_output  LeftPortType=input  RightPortType=output  PseudoPeriodic=off  Frequencies=[]  VectorFormat=inherit  Unit=W  AffineConversion=off
  PCC 10kV VI Sensor : ee_lib/Sensors & Transducers/Current and Voltage Sensor (Three-Phase)  port_option=ee.enum.threePhasePort.composite  vMeasurementType=ee.enum.vmeasurement.ll  outputUnit=ee.enum.unit.si  SRated=100e6 A*V  VRated=24e3 V  I_specify=off  I_priority=None  I=[0, 0, 0] A  I_nominal_specify=off  I_nominal_value=1  I_nominal_unit=A  V_specify=off  V_priority=None  V=[0, 0, 0] V  V_nominal_specify=off  V_nominal_value=1  V_nominal_unit=V
  PCC Current Local Terminator : Terminator
  PCC MeasurementBus : Mux
  PCC Voltage LL RMS : Fcn  Expr=sqrt((u(1)^2+u(2)^2+u(3)^2)/3)
  PCC iabc to Simulink : nesl_utility/PS-Simulink Converter  PhysicalDomain=network_engine_domain  SubClassName=ps_output  LeftPortType=input  RightPortType=output  PseudoPeriodic=off  Frequencies=[]  VectorFormat=inherit  Unit=A  AffineConversion=off
  PCC vabc to Simulink : nesl_utility/PS-Simulink Converter  PhysicalDomain=network_engine_domain  SubClassName=ps_output  LeftPortType=input  RightPortType=output  PseudoPeriodic=off  Frequencies=[]  VectorFormat=inherit  Unit=V  AffineConversion=off
  PV PCC Power Sensor : ee_lib/Sensors & Transducers/Power Sensor (Three-Phase)  port_option=ee.enum.threePhasePort.composite  load_type=ee.enum.passive.type_balanced.balanced  f0=60 Hz
  Q to Simulink : nesl_utility/PS-Simulink Converter  PhysicalDomain=network_engine_domain  SubClassName=ps_output  LeftPortType=input  RightPortType=output  PseudoPeriodic=off  Frequencies=[]  VectorFormat=inherit  Unit=W  AffineConversion=off
  T_PV_0p69_10kV : ee_lib/Passive/Transformers/Two-Winding Transformer (Three-Phase)  SRated=S1.transformer.S_VA A*V  FRated=S1.base.f_Hz Hz  Winding1Connection=ee.enum.windingconnection.Yg  VRated1=S1.pv.Vll_low_V V  Winding2Connection=ee.enum.windingconnection.Yg  VRated2=S1.pv.Vll_high_V V  CoreType=ee.enum.coretype.threelimb  pu_Rw1=S1.transformer.R_pu/2  pu_Rw2=S1.transformer.R_pu/2  leakage_reactance_option=ee.enum.transformer_leakage.exclude  pu_Xl1=0.05  pu_Xl2=0.05  magnetizing_resistance_option=ee.enum.transformer_magnetizingResistance.exclude  pu_Rm=500  magnetizing_reactance_option=ee.enum.transformer_magnetizingReactance.exclude  saturation_option=ee.enum.transformer_saturation.exclude  pu_Xm=500  current_data=[0, .002, 1, 2]  magnetic_flux_data=[0, 1.2, 1.5, 1.51]  pu_X0=0.5  i1_specify=off  i1_priority=None  i1=[0, 0, 0] A  i1_nominal_specify=off  i1_nominal_value=1  i1_nominal_unit=A  i2_specify=off  i2_priority=None  i2=[0, 0, 0] A  i2_nominal_specify=off  i2_nominal_value=1  i2_nominal_unit=A  phi_specify=off  phi_priority=None  phi=[0, 0, 0]  phi_nominal_specify=off  phi_nominal_value=1  phi_nominal_unit=1
  Conn1 : PMIOPort  Side=Right
  Conn2 : PMIOPort  Port=2  Side=Left
  tag scope: R21_PCCMeasurementBus=scoped
  wires:
  Q to Simulink/1 -> PCC MeasurementBus/3
  PCC vabc to Simulink/1 -> PCC MeasurementBus/1, PCC Voltage LL RMS/1
  PCC Voltage LL RMS/1 -> PCC MeasurementBus/4
  PCC iabc to Simulink/1 -> PCC Current Local Terminator/1
  P to Simulink/1 -> PCC MeasurementBus/2
  PCC MeasurementBus/1 -> [R21_PCCMeasurementBus]
  connections:
  PV PCC Power Sensor/RConn1 -- Conn1/RConn1
  PCC 10kV VI Sensor/RConn1 -- PCC vabc to Simulink/LConn1
  Conn2/RConn1 -- T_PV_0p69_10kV/LConn1
  PV PCC Power Sensor/LConn2 -- P to Simulink/LConn1
  PCC 10kV VI Sensor/RConn3 -- PV PCC Power Sensor/LConn1
  PV PCC Power Sensor/LConn3 -- Q to Simulink/LConn1
  PCC 10kV VI Sensor/RConn2 -- PCC iabc to Simulink/LConn1
  T_PV_0p69_10kV/RConn1 -- PCC 10kV VI Sensor/LConn1

== system BESS_PV_WIND_STAGE2_R1_with_scopes_r2024b/04 Wind-GFL Branch/01 Aerodynamic and MPPT Available Power ==
  WindCommandBus : Inport
  Available Power Limit : Saturate  UpperLimit=W1.wind.P_rated_W  LowerLimit=0
  Command Selector : Demux
  Dispatch Power Limit : Saturate  UpperLimit=W1.wind.P_rated_W  LowerLimit=0
  Enable Clamp : Saturate  UpperLimit=1  LowerLimit=0
  Mechanical Power Response : TransferFcn  Numerator=1  Denominator=[W1.wind.mechanical_tau_s 1]
  WindSourceBus : Mux
  WindSourceBus Out : Outport
  wires:
  WindSourceBus/1 -> WindSourceBus Out/1
  Enable Clamp/1 -> WindSourceBus/4
  Dispatch Power Limit/1 -> WindSourceBus/2
  Mechanical Power Response/1 -> WindSourceBus/1
  Available Power Limit/1 -> Mechanical Power Response/1
  Command Selector/4 -> Enable Clamp/1
  Command Selector/3 -> WindSourceBus/3
  Command Selector/2 -> Dispatch Power Limit/1
  Command Selector/1 -> Available Power Limit/1
  WindCommandBus/1 -> Command Selector/1

== system BESS_PV_WIND_STAGE2_R1_with_scopes_r2024b/04 Wind-GFL Branch/02 DC Energy Buffer and MSC Equivalent ==
  WindSourceBus : Inport
  Available versus Dispatch : MinMax  Inputs=2
  DC Energy Buffer : TransferFcn  Numerator=1  Denominator=[W1.dc.buffer_tau_s 1]
  DC Energy Delta : Integrator
  DC Power Imbalance : Sum  Inputs=+-
  DC Voltage from Energy : Fcn  Expr=sqrt(abs(2*u/W1.dc.C_equiv_F))
  MPPT Capture pu : Gain  Gain=1/W1.wind.P_rated_W
  MSC Power Ramp : RateLimiter  RisingSlewLimit=W1.wind.source_ramp_up_Wps  FallingSlewLimit=W1.wind.source_ramp_down_Wps  SampleTimeMode=inherited
  Nominal DC Energy : Bias  Bias=W1.dc.energy_buffer_J  SaturateOnIntegerOverflow=off
  PCS CommandBus : Mux  Inputs=3
  Source Selector : Demux
  Source StatusBus : Mux  Inputs=5
  PCS CommandBus Out : Outport
  Source StatusBus Out : Outport  Port=2
  wires:
  MPPT Capture pu/1 -> Source StatusBus/5
  PCS CommandBus/1 -> PCS CommandBus Out/1
  WindSourceBus/1 -> Source Selector/1
  Source Selector/3 -> PCS CommandBus/2
  Source Selector/1 -> Source StatusBus/1, Available versus Dispatch/1, MPPT Capture pu/1
  Source Selector/4 -> PCS CommandBus/3
  Source Selector/2 -> Source StatusBus/2, Available versus Dispatch/2
  DC Energy Buffer/1 -> DC Power Imbalance/2, PCS CommandBus/1, Source StatusBus/3
  MSC Power Ramp/1 -> DC Energy Buffer/1
  Available versus Dispatch/1 -> DC Power Imbalance/1, MSC Power Ramp/1
  DC Power Imbalance/1 -> DC Energy Delta/1
  Nominal DC Energy/1 -> DC Voltage from Energy/1
  DC Energy Delta/1 -> Nominal DC Energy/1
  DC Voltage from Energy/1 -> Source StatusBus/4
  Source StatusBus/1 -> Source StatusBus Out/1

== system BESS_PV_WIND_STAGE2_R1_with_scopes_r2024b/04 Wind-GFL Branch/03 GFL PCS ==
  CommandBus : Inport
  01 Secondary Control : Subsystem
  02 Primary Converter and Filter : Subsystem
  AC_690V : PMIOPort  Side=Right
  StatusBus : Outport
  wires:
  CommandBus/1 -> 01 Secondary Control/1(In1)
  01 Secondary Control/1(Out4) -> StatusBus/1
  connections:
  02 Primary Converter and Filter/RConn1 -- AC_690V/RConn1

== system BESS_PV_WIND_STAGE2_R1_with_scopes_r2024b/04 Wind-GFL Branch/04 Step-up and PCC ==
  P to Simulink : nesl_utility/PS-Simulink Converter  PhysicalDomain=network_engine_domain  SubClassName=ps_output  LeftPortType=input  RightPortType=output  PseudoPeriodic=off  Frequencies=[]  VectorFormat=inherit  Unit=W  AffineConversion=off
  PCC 10kV VI Sensor : ee_lib/Sensors & Transducers/Current and Voltage Sensor (Three-Phase)  port_option=ee.enum.threePhasePort.composite  vMeasurementType=ee.enum.vmeasurement.ll  outputUnit=ee.enum.unit.si  SRated=100e6 A*V  VRated=24e3 V  I_specify=off  I_priority=None  I=[0, 0, 0] A  I_nominal_specify=off  I_nominal_value=1  I_nominal_unit=A  V_specify=off  V_priority=None  V=[0, 0, 0] V  V_nominal_specify=off  V_nominal_value=1  V_nominal_unit=V
  PCC Current Local Terminator : Terminator
  PCC MeasurementBus : Mux
  PCC Voltage LL RMS : Fcn  Expr=sqrt((u(1)^2+u(2)^2+u(3)^2)/3)
  PCC iabc to Simulink : nesl_utility/PS-Simulink Converter  PhysicalDomain=network_engine_domain  SubClassName=ps_output  LeftPortType=input  RightPortType=output  PseudoPeriodic=off  Frequencies=[]  VectorFormat=inherit  Unit=A  AffineConversion=off
  PCC vabc to Simulink : nesl_utility/PS-Simulink Converter  PhysicalDomain=network_engine_domain  SubClassName=ps_output  LeftPortType=input  RightPortType=output  PseudoPeriodic=off  Frequencies=[]  VectorFormat=inherit  Unit=V  AffineConversion=off
  Q to Simulink : nesl_utility/PS-Simulink Converter  PhysicalDomain=network_engine_domain  SubClassName=ps_output  LeftPortType=input  RightPortType=output  PseudoPeriodic=off  Frequencies=[]  VectorFormat=inherit  Unit=W  AffineConversion=off
  T_Wind_0p69_10kV : ee_lib/Passive/Transformers/Two-Winding Transformer (Three-Phase)  SRated=S1.transformer.S_VA A*V  FRated=S1.base.f_Hz Hz  Winding1Connection=ee.enum.windingconnection.Yg  VRated1=S1.pv.Vll_low_V V  Winding2Connection=ee.enum.windingconnection.Yg  VRated2=S1.pv.Vll_high_V V  CoreType=ee.enum.coretype.threelimb  pu_Rw1=S1.transformer.R_pu/2  pu_Rw2=S1.transformer.R_pu/2  leakage_reactance_option=ee.enum.transformer_leakage.exclude  pu_Xl1=0.05  pu_Xl2=0.05  magnetizing_resistance_option=ee.enum.transformer_magnetizingResistance.exclude  pu_Rm=500  magnetizing_reactance_option=ee.enum.transformer_magnetizingReactance.exclude  saturation_option=ee.enum.transformer_saturation.exclude  pu_Xm=500  current_data=[0, .002, 1, 2]  magnetic_flux_data=[0, 1.2, 1.5, 1.51]  pu_X0=0.5  i1_specify=off  i1_priority=None  i1=[0, 0, 0] A  i1_nominal_specify=off  i1_nominal_value=1  i1_nominal_unit=A  i2_specify=off  i2_priority=None  i2=[0, 0, 0] A  i2_nominal_specify=off  i2_nominal_value=1  i2_nominal_unit=A  phi_specify=off  phi_priority=None  phi=[0, 0, 0]  phi_nominal_specify=off  phi_nominal_value=1  phi_nominal_unit=1
  Wind PCC Power Sensor : ee_lib/Sensors & Transducers/Power Sensor (Three-Phase)  port_option=ee.enum.threePhasePort.composite  load_type=ee.enum.passive.type_balanced.balanced  f0=60 Hz
  Conn1 : PMIOPort  Side=Right
  Conn2 : PMIOPort  Port=2  Side=Left
  tag scope: WIND1_PCCMeasurementBus=scoped
  wires:
  PCC iabc to Simulink/1 -> PCC Current Local Terminator/1
  PCC vabc to Simulink/1 -> PCC MeasurementBus/1, PCC Voltage LL RMS/1
  PCC Voltage LL RMS/1 -> PCC MeasurementBus/4
  P to Simulink/1 -> PCC MeasurementBus/2
  Q to Simulink/1 -> PCC MeasurementBus/3
  PCC MeasurementBus/1 -> [WIND1_PCCMeasurementBus]
  connections:
  Wind PCC Power Sensor/RConn1 -- Conn1/RConn1
  Conn2/RConn1 -- T_Wind_0p69_10kV/LConn1
  PCC 10kV VI Sensor/RConn2 -- PCC iabc to Simulink/LConn1
  T_Wind_0p69_10kV/RConn1 -- PCC 10kV VI Sensor/LConn1
  PCC 10kV VI Sensor/RConn3 -- Wind PCC Power Sensor/LConn1
  PCC 10kV VI Sensor/RConn1 -- PCC vabc to Simulink/LConn1
  Wind PCC Power Sensor/LConn2 -- P to Simulink/LConn1
  Wind PCC Power Sensor/LConn3 -- Q to Simulink/LConn1

== system BESS_PV_WIND_STAGE2_R1_with_scopes_r2024b/06 Supervision and Results/01 PV Command Profile ==
  CommandBus : Mux  Inputs=3
  Enable : Sum  Inputs=+++
  Enable Base : Constant
  Enable Off : Step  Time=10  After=0  SampleTime=0
  Enable On : Step  Time=11  After=0  SampleTime=0
  P Base Limit : Saturate  UpperLimit=5000000  LowerLimit=0
  P Command : Sum
  P Increment : Step  Time=0.30  After=0  SampleTime=0
  P Soft Start : simulink/Sources/Ramp  slope=S1.pv.P_ramp_W_per_s  start=0  InitialOutput=0
  Q Base Command : Constant  Value=2421610.524189263
  Q Command : Sum
  Q Increment : Step  Time=0.30  After=0  SampleTime=0
  CommandBus Out : Outport
  wires:
  Enable/1 -> CommandBus/3
  Enable On/1 -> Enable/3
  Enable Off/1 -> Enable/2
  Enable Base/1 -> Enable/1
  CommandBus/1 -> CommandBus Out/1
  Q Command/1 -> CommandBus/2
  P Command/1 -> CommandBus/1
  Q Increment/1 -> Q Command/2
  P Base Limit/1 -> P Command/1
  P Soft Start/1 -> P Base Limit/1
  Q Base Command/1 -> Q Command/1
  P Increment/1 -> P Command/2

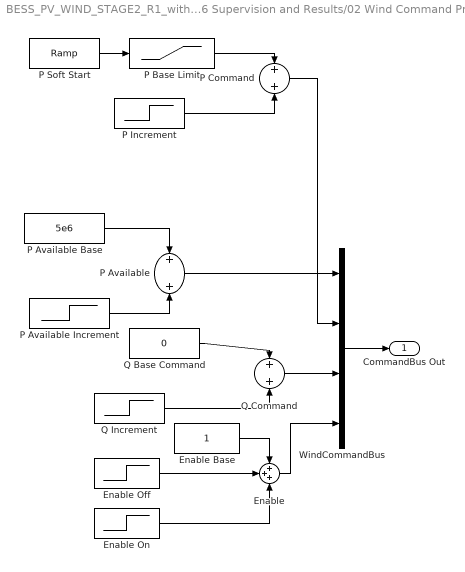
== system BESS_PV_WIND_STAGE2_R1_with_scopes_r2024b/06 Supervision and Results/02 Wind Command Profile ==
  Enable : Sum  Inputs=+++
  Enable Base : Constant
  Enable Off : Step  Time=10  After=0  SampleTime=0
  Enable On : Step  Time=11  After=0  SampleTime=0
  P Available : Sum
  P Available Base : Constant  Value=5e6
  P Available Increment : Step  Time=0.30  After=0  SampleTime=0
  P Base Limit : Saturate  UpperLimit=5e6  LowerLimit=0
  P Command : Sum
  P Increment : Step  Time=0.30  After=0  SampleTime=0
  P Soft Start : simulink/Sources/Ramp  slope=S1.pv.P_ramp_W_per_s  start=0  InitialOutput=0
  Q Base Command : Constant  Value=0
  Q Command : Sum
  Q Increment : Step  Time=0.30  After=0  SampleTime=0
  WindCommandBus : Mux
  CommandBus Out : Outport
  wires:
  Enable/1 -> WindCommandBus/4
  Q Command/1 -> WindCommandBus/3
  P Command/1 -> WindCommandBus/2
  P Available/1 -> WindCommandBus/1
  P Available Increment/1 -> P Available/2
  P Available Base/1 -> P Available/1
  Enable On/1 -> Enable/3
  Enable Off/1 -> Enable/2
  Enable Base/1 -> Enable/1
  WindCommandBus/1 -> CommandBus Out/1
  Q Increment/1 -> Q Command/2
  Q Base Command/1 -> Q Command/1
  P Increment/1 -> P Command/2
  P Base Limit/1 -> P Command/1
  P Soft Start/1 -> P Base Limit/1
